simulink model "LabA_LinearizedBot"  (R2026b)
settings: Solver=ode14x  StopTime=5  FixedStep=0.001  RelTol=1e-2  EnableMultiTasking=on
values from neighbouring files (symbols this model uses):
  A = [0, 1, 0, 0 ... (first row only)    [LabA_equations.m]    (also in LabA_parameters.mat = [0 0 0 0 1 0.0716665297455 0 0.0185556406229 0 0.01784481592; LabB_ObserverAndControllerOverSimulator_Continuous_Parameters.m = 1.0e+03 * [; matlab.mat = [0 0 0 0 1 -435.034344762 0 1903.43949265 0 -6.0990753006 0 )
  Bd = [0,           0 ... (first row only)    [LabA_equations.m]    (also in LabB_ObserverOverSimulator_Discrete_Parameters.m = [)
  Cf = eye(4)    [LabA_equations.m]
  D_bd = zeros(4, 2)    [LabA_equations.m]
  Kd_val = (alpha2 - a2) / b1    [LabA_equations.m]
  Ki_val = (alpha0 - a0) / b1    [LabA_equations.m]
  Kp_val = (alpha1 - a1) / b1    [LabA_equations.m]
undefined symbols (not defined in the file or in its folder): sigbuilder_block
libraries: cstblocks_lti x1, slpidlib x1
settings Model: Creator=The MathWorks Inc.  LastModifiedBy=holyk
settings DataIOCC: LimitDataPoints=on  ReturnWorkspaceOutputs=off  SaveFormat=Array  SignalLoggingName=logsOut
settings OptimizationCC: EfficientMapNaN2IntZero=off  MemsetInitFltsAndDblsToZero=off
settings DebuggingCC: ArithmeticOperatorsInVariantConditions=warning  FcnCallInpInsideContextMsg=warning  MergeDetectMultiDrivingBlocksExec=none  SFExecutionAtInitializationDiag=none  SFNoUnconditionalDefaultTransitionDiag=warning  SFUnexpectedBacktrackingDiag=warning  SignalResolutionControl=TryResolveAllWithWarning  StateNameClashWarn=warning  UnderspecifiedInitializationDetection=Classic
settings HardwareCC: TargetEndianess=LittleEndian  TargetHWDeviceType=Intel->x86-64  TargetIntDivRoundTo=Zero
settings ModelReferenceCC: PropagateSignalLabelsOutOfModel=off
settings SFSimCC: CustomCodeUndefinedFunction=UseInterfaceOnly  SimUseLocalCustomCode=off
settings RTWCC: Description=Simulink Desktop Real-Time  RTWCompilerOptimization=on  RTWUseLocalCustomCode=off  SystemTargetFile=sldrt.tlc  TemplateMakefile=sldrt.tmf
settings CodeAppCC: StateflowObjectComments=on
settings SimulinkDesktopRealTimeCC: TargetLangStandard=C89/C90 (ANSI)  TargetPreCompLibLocation=C:\Program Files\MATLAB\R2017a\toolbox\sldrt\lib\win64
settings ConfigComp: CovExternalEMLEnable=off  CovSFcnEnable=off  CovSaveCumulativeToWorkspaceVar=on  CovSaveSingleToWorkspaceVar=on

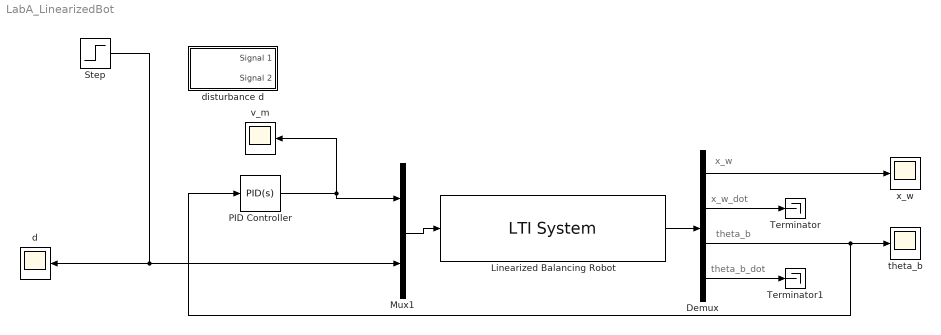
== system LabA_LinearizedBot ==
  note: x_w_dot
  note: x_w
  note: theta_b
  note: theta_b_dot
  Demux : Demux
  Linearized Balancing Robot : cstblocks_lti/LTI System  sys=ss(A, Bd, Cf, D_bd)  IC=[0 0 0*pi/180 0]  PadeOrder=0
  Mux1 : Mux  Inputs=2
  "PID Controller " : slpidlib/PID Controller  Controller=PID  Form=Parallel  TimeDomain=Continuous-time  UseExternalTs=off  SampleTime=-1  IntegratorMethod=Forward Euler  FilterMethod=Forward Euler  ControllerParametersSource=internal  P=-Kp_val  I=-Ki_val  UseKiTs=off  D=-Kd_val  UseExternalDerivativeSource=off  N=100000  UseFilter=on  TunerSelectOption=Transfer Function Based (PID Tuner App)  InitialConditionSource=internal  InitialConditionForIntegrator=0  InitialConditionForFilter=0  DifferentiatorICPrevScaledInput=0  ExternalReset=none  TrackingMode=off  Kt=1  LimitOutput=off  SatLimitsSource=internal  UpperSaturationLimit=inf  LowerSaturationLimit=-inf  LinearizeAsGain=on  AntiWindupMode=none  Kb=1  LimitIntegrator=off  UpperIntegratorSaturationLimit=inf  LowerIntegratorSaturationLimit=-inf  POutMin=[]  POutMax=[]  IOutMin=[]  IOutMax=[]  DOutMin=[]  DOutMax=[]  NOutMin=[]  NOutMax=[]  SumOutMin=[]  SumOutMax=[]  SaturationOutMin=[]  SaturationOutMax=[]  PParamMin=[]  PParamMax=[]  IParamMin=[]  IParamMax=[]  DParamMin=[]  DParamMax=[]  NParamMin=[]  NParamMax=[]  KbParamMin=[]  KbParamMax=[]  KtParamMin=[]  KtParamMax=[]  KbOutMin=[]  KbOutMax=[]  KtOutMin=[]  KtOutMax=[]  IntegratorOutMin=[]  IntegratorOutMax=[]  FilterOutMin=[]  FilterOutMax=[]  SumI1OutMin=[]  SumI1OutMax=[]  SumI2OutMin=[]  SumI2OutMax=[]  SumI3OutMin=[]  SumI3OutMax=[]  SumI4OutMin=[]  SumI4OutMax=[]  SumDOutMin=[]  SumDOutMax=[]  DifferentiatorOutMin=[]  DifferentiatorOutMax=[]  FilterDiffOutCoefMin=[]  FilterDiffOutCoefMax=[]  ReciprocalOutMin=[]  ReciprocalOutMax=[]  SumDenOutMin=[]  SumDenOutMax=[]  SumNumOutMin=[]  SumNumOutMax=[]  DivideOutMin=[]  DivideOutMax=[]  UdiffTsProdOutMin=[]  UdiffTsProdOutMax=[]  NTsProdOutMin=[]  NTsProdOutMax=[]  UintegralTsProdOutMin=[]  UintegralTsProdOutMax=[]  UngainTsProdOutMin=[]  UngainTsProdOutMax=[]  ClampingZeroOutDataTypeStr=Inherit: Inherit via back propagation  ClampingZeroOutMin=[]  ClampingZeroOutMax=[]  FilterDenConstantOutDataTypeStr=Inherit: Inherit via back propagation  FilterDenConstantOutMin=[]  FilterDenConstantOutMax=[]  PCopyOutDataTypeStr=Inherit: Inherit via back propagation  PCopyOutMin=[]  PCopyOutMax=[]  NCopyOutDataTypeStr=Inherit: Inherit via back propagation  NCopyOutMin=[]  NCopyOutMax=[]  IntegratorContinuousStateAttributes=''  IntegratorStateMustResolveToSignalObject=off  IntegratorRTWStateStorageClass=Auto  FilterContinuousStateAttributes=''  FilterStateMustResolveToSignalObject=off  FilterRTWStateStorageClass=Auto  ParallelPVariant=InternalParameters  IdealPVariant=Disabled  IVariant=InternalParameters  DVariant=InternalParameters  IntegratorVariant=Continuous  SatVariant=Disabled  AWVariant=Passthrough  PCopyVariant=Disabled  TRVariant=Disabled  FdbkBlocksVariant=Forward  IdealPFdbkVariant=Disabled  SatFdbkVariant=Disabled  DerivativeFilterVariant=ContFilter  NVariant=InternalParameters  NCopyVariant=Disabled  FilterICVariant=InternalICsFilter  IntegratorICVariant=InternalICs  ExternalResetVariant=Disabled  TRSumVariant=Passthrough  SumFdbkVariant=Disabled  SumVariant=Sum_PID  TsampFilterVariant=InternalTs  TsampNgainVariant=Passthrough  TsampIntegralVariant=Disabled_SignalSpec  ExternalSaturationOutDataTypeStr=Inherit: Same as second input  DerivativeSourceVariant=ErrorSignal  PreIntVariant=InternalPreInt
  Step : Step  Time=0.1  InitialValue=0.1  FinalValue=0  SampleTime=0
  Terminator : Terminator
  Terminator1 : Terminator
  d : Scope
      settings: ActiveDisplayYMinimum=-0.012499999999999997  ActiveDisplayYMaximum=0.1125  DataLoggingVariableName=d
  disturbance d : Subsystem  Tag=STV Subsys  LoadFcn=sigbuilder_block('load');  StartFcn=sigbuilder_block('start');  StopFcn=sigbuilder_block('stop');  ClipboardFcn=sigbuilder_block('clipboard');  mask(Sigbuilder block){tuvar=[0:10]}
      mask help: Simulink:masks:SigbuilderBlock_MD
      mask init:
      | if ~strcmp(get_param(bdroot(gcbh),'SimulationStatus'),'stopped') tuvar = sigbuilder_block('maskInit'); end
      settings: CopyFcn=sigbuilder_block('copy');  DeleteFcn=sigbuilder_block('delete');  ModelCloseFcn=sigbuilder_block('modelClose');  PreSaveFcn=sigbuilder_block('preSave');  PauseFcn=sigbuilder_block('pause');  ContinueFcn=sigbuilder_block('continue');  NameChangeFcn=sigbuilder_block('namechange');  OpenFcn=sigbuilder_block('open',[414.75 146.25 539.25 335.25 ]);  CloseFcn=sigbuilder_block('close');
      mask Display: plot(0, 0, 100, 100,[2, 2, 32, 32, 2], [68, 8, 8, 68, 68],[32, 2], [38, 38], [32, 19, 2],[53, 60, 44], [32, 17, 17, 2],[16, 16, 31, 31]);txt = getActiveGroup(gcbh);text(2, 100, txt,'verticalAlignment', 'top');
  theta_b : Scope
      settings: ActiveDisplayYMinimum=-0.003  ActiveDisplayYMaximum=0.018  DataLoggingVariableName=theta_b
  v_m : Scope
      settings: ActiveDisplayYMinimum=-0.13575589824774428  ActiveDisplayYMaximum=1.2218030842296987  DataLoggingVariableName=v_m
  x_w : Scope
      settings: ActiveDisplayYMinimum=-0.03064913852739605  ActiveDisplayYMaximum=0.27584224674656449  DataLoggingVariableName=x_w
  wires:
  Mux1/1 -> Linearized Balancing Robot/1
  Linearized Balancing Robot/1 -> Demux/1
  Demux/1 -> x_w/1
  Demux/3 -> theta_b/1, "PID Controller "/1
  "PID Controller "/1 -> v_m/1, Mux1/1
  Demux/4 -> Terminator1/1
  Demux/2 -> Terminator/1
  Step/1 -> Mux1/2, d/1

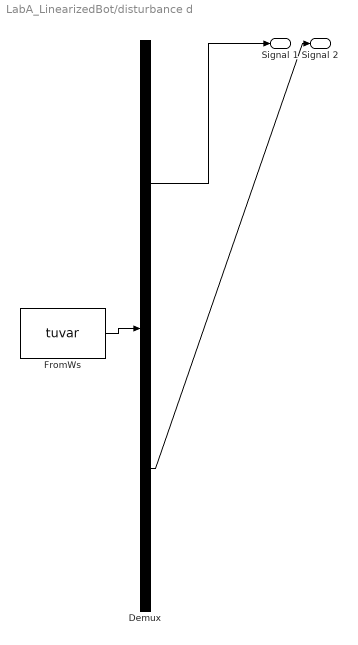
== system LabA_LinearizedBot/disturbance d ==
  Demux : Demux  Tag=STV Demux  Outputs=2
      settings: DisplayOption=none
  FromWs : FromWorkspace  Tag=STV FromWs  VariableName=tuvar
      SigBuilderData=|
      | common.afterFinalStr = 'Extrapolate'
      | common.sampleTime = 0
      | dataSet.timeRange = [0 10]
      | dataSet.name = 'Group 1'
      | sbobj.Groups.Name = 'Group 1'
      | sbobj.Groups.Signals(1).Name = 'Signal 1'
      | sbobj.Groups.Signals(1).XData = [0 0.1 0.1 10]
      | sbobj.Groups.Signals(1).YData = [0.02 0.02 0 0]
      | sbobj.Groups.Signals(2).Name = 'Signal 2'
      | sbobj.Groups.Signals(2).XData = [0 10]
      | sbobj.Groups.Signals(2).YData = [0 0]
  Signal 1 : Outport  Tag=STV Outport
  Signal 2 : Outport  Tag=STV Outport  Port=2
  wires:
  Demux/1 -> Signal 1/1
  FromWs/1 -> Demux/1
  Demux/2 -> Signal 2/1
